simulink model "rocket_sim"  (R2023a)
settings: Solver=VariableStepAuto  StartTime=0.0  StopTime=480  RelTol=1e-3
undefined symbols (not defined in the file or in its folder): Earth, WGS84
libraries: simulink x55, slpidlib x10, aerolibconvert2 x7, matrix_library x4, aerolibasang x3, aerolibtransform2 x2, aerolibatmos2 x2, shared6dof x1, sharedtransform x1
(part 1 of 3)
settings Model: Creator=Administrator  LastModifiedBy=ROG

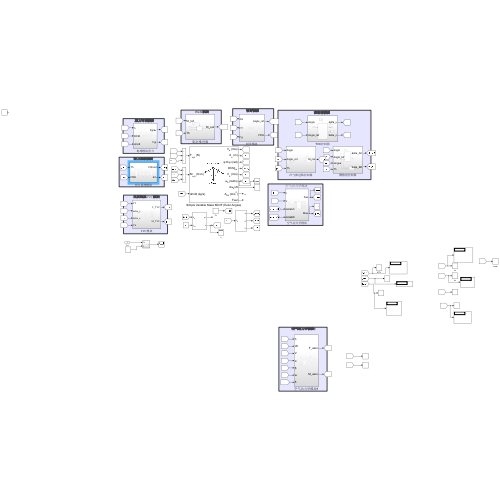
[thumbnail: Simulink's stored preview of the top-level diagram]
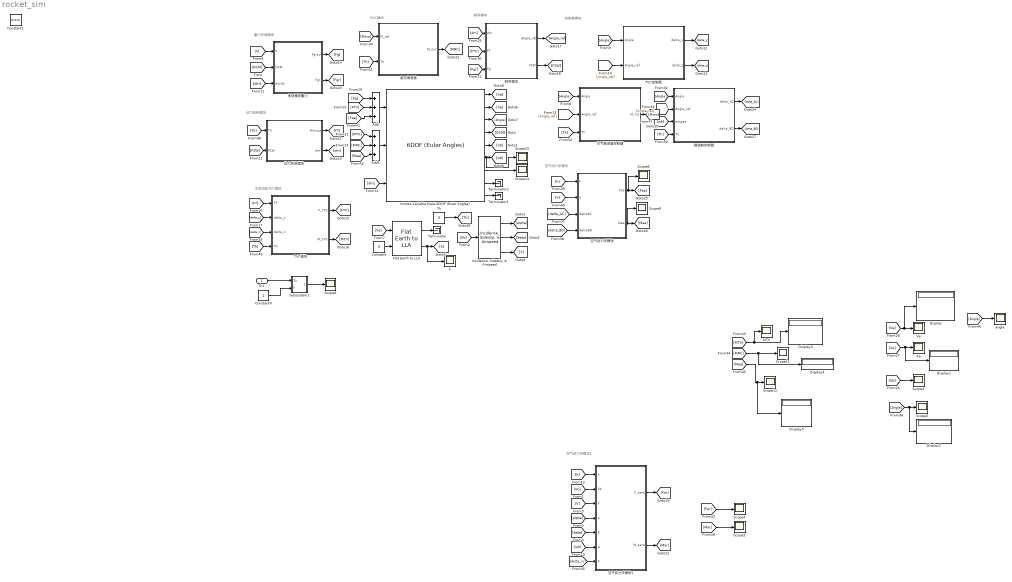
== system rocket_sim ==
  note: 空气动力学模块
  note: 控制器模块
  note: 空气动力学模块1
  note: 制导模块
  note: RCS模块
  note: 动力系统模块
  note: 重力环境模块
  note: 主发动机TVC模块
  Th1 : Inport
  Add : Sum  Inputs=+++
  Add1 : Sum  Inputs=+++
  Constant : Constant  Value=0
  Constant1 : Constant  Value=[0;0;0]
  Constant4 : Constant
  Display{,1..5} (6 alike) : Display
  Flat Earth to LLA : aerolibtransform2/Flat Earth to LLA  units=Metric (MKS)  ptype=Earth (WGS84)  F=1/298.257223563  R=6378137  refPosPort=off  LL0=[0 10]  psi=0
  "Incidence, Sideslip, & Airspeed" : aerolibasang/Incidence, Sideslip, & Airspeed
  MTV : Scope
  Scope{2..6,8..9,11..12,14..15} (11 alike) : Scope
  Simple Variable Mass 6DOF (Euler Angles) : shared6dof/6DOF (Euler Angles)  units=Metric (MKS)  mtype=Simple Variable  rep=Euler Angles  xme_0=[0 0 0]  Vm_0=[0 0 0]  eul_0=[0 pi/2 0]  pm_0=[0 0 0]  mass_0=549e3  mass_e=22.2e3  mass_f=549e3  inertia=eye(3)  inertia_e=6.06e4*eye(3)  inertia_f=149.9e4*eye(3)  k_quat=1.0  vre_flag=off  abi_flag=off  aMode=0  xme_statename=''  Vm_statename=''  eul_statename=''  quat_statename=''  pm_statename=''  mass_statename=''
      settings: LibrarySourceBlock=aerolib6dof2/Simple Variable Mass 6DOF (Euler Angles)
  Subsystem1 : Subsystem
  TVC控制器 : Subsystem
  TVC模块 : Subsystem
  Terminator : Terminator
  Terminator1 : Terminator
  Terminator2 : Terminator
  Th : Constant  Value=0
  Ve : Scope
  Xe : Scope
  angle : Scope
  h : Scope
  冷气推进器控制器 : Subsystem
  制导模块 : Subsystem
  动力系统模块 : Subsystem
  地球模块重力 : Subsystem
  姿态推进器 : Subsystem
  栅格舵控制器 : Subsystem
  空气动力学模块 : Subsystem
  空气动力学模块1 : Subsystem
  wires:
  [h] -> 地球模块重力/1(h)
  Simple Variable Mass 6DOF (Euler Angles)/4 -> [DCM]
  [DCM] -> 地球模块重力/2(DCM)
  Simple Variable Mass 6DOF (Euler Angles)/5 -> [Vb]
  [Vb] -> 空气动力学模块1/2(Vb)
  [Vb] -> "Incidence, Sideslip, & Airspeed"/1
  "Incidence, Sideslip, & Airspeed"/1 -> [alpha]
  "Incidence, Sideslip, & Airspeed"/2 -> [beta]
  "Incidence, Sideslip, & Airspeed"/3 -> [V]
  [alpha] -> 空气动力学模块1/4(α)
  [beta] -> 空气动力学模块1/5(β)
  [V] -> 空气动力学模块1/3(V)
  Flat Earth to LLA/1 -> Terminator/1
  Flat Earth to LLA/2 -> h/1, [h]
  Constant/1 -> Flat Earth to LLA/2
  Simple Variable Mass 6DOF (Euler Angles)/2 -> [Xe]
  [Xe] -> Flat Earth to LLA/1
  Simple Variable Mass 6DOF (Euler Angles)/3 -> [Angle]
  Simple Variable Mass 6DOF (Euler Angles)/1 -> [Ve]
  Simple Variable Mass 6DOF (Euler Angles)/6 -> Scope15/1, [wb]
  动力系统模块/2(dm) -> [dm]
  [dm] -> 地球模块重力/3(dm/dt)
  [dm] -> Simple Variable Mass 6DOF (Euler Angles)/3
  [h] -> 空气动力学模块1/1(h)
  [FT] -> TVC模块/1(FT)
  [delta_y] -> TVC模块/2(delta_y)
  [delta_z] -> TVC模块/3(delta_z)
  Add/1 -> Simple Variable Mass 6DOF (Euler Angles)/1
  Add1/1 -> Simple Variable Mass 6DOF (Euler Angles)/2
  地球模块重力/1(Fgrav) -> [Fg]
  [Fg] -> Add/1
  TVC模块/1(F_TVC) -> [FTV]
  TVC模块/2(M_TVC) -> [MTV]
  [FTV] -> Add/2
  [MTV] -> Add1/1
  动力系统模块/1(Fthrust) -> [FT]
  [wb] -> 空气动力学模块1/6(w)
  制导模块/1(Angle_ref) -> [Angle_ref]
  Simple Variable Mass 6DOF (Euler Angles)/9 -> Terminator1/1
  Simple Variable Mass 6DOF (Euler Angles)/8 -> Terminator2/1
  [Angle] -> TVC控制器/1(Angle)
  [Angle_ref] -> TVC控制器/2(Angle_ref)
  TVC控制器/2(delta_z) -> [delta_z]
  TVC控制器/1(delta_y) -> [delta_y]
  制导模块/2(FSW) -> [FSW]
  [FSW] -> 动力系统模块/2(FSW)
  空气动力学模块1/1(F_aero) -> [Far]
  空气动力学模块1/2(M_aero) -> [Mar]
  姿态推进器/1(M_out) -> [MRC]
  [Ve] -> Display/1, Ve/1
  [Xe] -> Display1/1, Xe/1
  [Vb] -> Scope2/1
  [MRC] -> Add1/2
  [dm] -> 制导模块/1(dm)
  [FTV] -> 制导模块/2(FT)
  [Fgr] -> 制导模块/3(Fg)
  地球模块重力/2(Fgr) -> [Fgr]
  [delta_ru] -> 空气动力学模块1/7(δ)
  [Angle] -> Display2/1, Scope3/1
  [Far] -> Scope4/1
  [Mar] -> Scope5/1
  冷气推进器控制器/1(M_rcs) -> [Mrcs]
  栅格舵控制器/1(delta_AC) -> [delta_AC]
  [Mrcs] -> 姿态推进器/1(M_ref)
  [Angle_ref] -> 冷气推进器控制器/2(Angle_ref)
  [Angle] -> 冷气推进器控制器/1(Angle)
  [Angle_ref] -> 栅格舵控制器/2(Angle_ref)
  [Angle] -> 栅格舵控制器/1(Angle)
  Constant4/1 -> Subsystem1/2(F)
  Th1/1 -> Subsystem1/1(Th)
  Subsystem1/1(Out1) -> Scope6/1
  [Faa] -> Add/3
  [Maa] -> Add1/3
  空气动力学模块/1(Faa) -> Scope8/1, [Faa]
  空气动力学模块/2(Maa) -> Scope9/1, [Maa]
  [h] -> 空气动力学模块/1(h)
  [V] -> 空气动力学模块/2(V)
  栅格舵控制器/2(delta_BD) -> [delta_BD]
  [MTV] -> MTV/1, Display3/1
  [MRC] -> Display4/1, Scope11/1
  [Maa] -> Display5/1, Scope12/1
  [delta_AC] -> 空气动力学模块/3(deltaAC)
  [delta_BD] -> 空气动力学模块/4(deltaBD)
  [Angle] -> angle/1
  Simple Variable Mass 6DOF (Euler Angles)/7 -> Scope14/1
  [wb] -> 栅格舵控制器/3(omgea)
  Th/1 -> [Th]
  [Th] -> 动力系统模块/1(Th)
  [Th] -> TVC模块/4(Th)
  [Th] -> 栅格舵控制器/4(Th)
  [Th] -> 姿态推进器/2(Th)
  [Th] -> 冷气推进器控制器/3(Th)

== system rocket_sim/Subsystem1 ==
  Th : Inport
  F : Inport  Port=2
  Constant4 : Constant  Value=0
  Step1 : Step  Time=200  SampleTime=0
  Step2 : Step  Time=480  SampleTime=0
  Switch : Switch  Criteria=u2 > Threshold  SaturateOnIntegerOverflow=off  InputSameDT=off
  Switch1 : Switch  Criteria=u2 > Threshold  SaturateOnIntegerOverflow=off  InputSameDT=off
  Switch2 : Switch  Criteria=u2 > Threshold  SaturateOnIntegerOverflow=off  InputSameDT=off
  故障 : Subsystem
  退化 : Subsystem
  Out1 : Outport
  wires:
  F/1 -> Switch2/2
  退化/1(Out1) -> Switch1/3, Switch/1
  Switch1/1 -> Switch/3
  Constant4/1 -> Switch2/1
  Switch2/1 -> Switch1/2
  Th/1 -> 故障/1(Th1), 退化/1(Th)
  Step2/1 -> Switch/2
  Switch/1 -> Out1/1
  Step1/1 -> Switch2/3
  故障/1(Out1) -> Switch1/1

== system rocket_sim/TVC控制器 ==
  Angle : Inport
  Angle_ref : Inport  Port=2
  Constant : Constant
  Scope : Scope
  Scope1 : Scope
  Subsystem : Subsystem
  delta_y : Outport
  delta_z : Outport  Port=2
  wires:
  Angle/1 -> Subsystem/1(Angle)
  Angle_ref/1 -> Subsystem/2(Angle_ref)
  Subsystem/1(delta_z) -> Scope/1, delta_z/1
  Subsystem/2(delta_y) -> Scope1/1, delta_y/1
  Constant/1 -> Subsystem/Enable

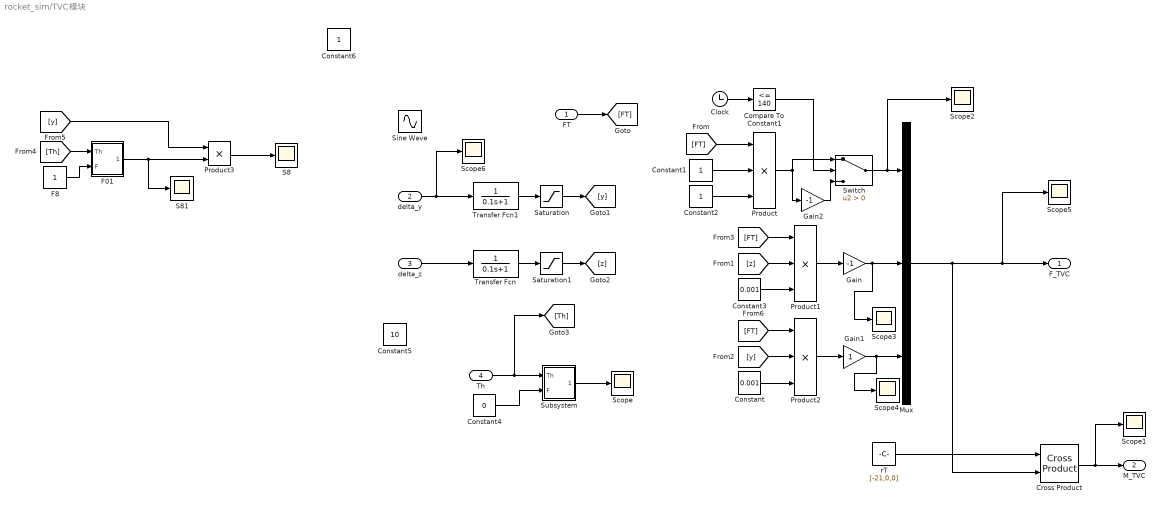
== system rocket_sim/TVC模块 ==
  FT : Inport
  delta_y : Inport  Port=2
  delta_z : Inport  Port=3
  Th : Inport  Port=4
  Clock : Clock
  Compare To Constant1 : simulink/Logic and Bit Operations/Compare To Constant  relop=<=  const=140  OutDataTypeStr=boolean
  Constant : Constant  Value=0.001
  Constant1 : Constant
  Constant2 : Constant
  Constant3 : Constant  Value=0.001
  Constant4 : Constant  Value=0
  Constant5 : Constant  Value=10
  Constant6 : Constant
  Cross Product : matrix_library/Cross Product
  F01 : Subsystem
  F8 : Constant
  Gain : Gain  Gain=-1
  Gain1 : Gain
  Gain2 : Gain  Gain=-1
  Mux : Mux  Inputs=3
  Product : Product  Inputs=3
  Product1 : Product  Inputs=3
  Product2 : Product  Inputs=3
  Product3 : Product
  S8 : Scope
  S81 : Scope
  Saturation : Saturate  UpperLimit=3  LowerLimit=-3
  Saturation1 : Saturate  UpperLimit=3  LowerLimit=-3
  Scope{,1..6} (7 alike) : Scope
  Sine Wave : Sin  SampleTime=0
  Subsystem : Subsystem
  Switch : Switch  Criteria=u2 > Threshold  SaturateOnIntegerOverflow=off  InputSameDT=off
  Transfer Fcn : TransferFcn  Denominator=[0.1 1]
  Transfer Fcn1 : TransferFcn  Denominator=[0.1 1]
  rT : Constant  Value=[-21,0,0]
  F_TVC : Outport
  M_TVC : Outport  Port=2
  wires:
  FT/1 -> [FT]
  [FT] -> Product/1
  Constant2/1 -> Product/3
  [FT] -> Product1/1
  [FT] -> Product2/1
  Constant/1 -> Product2/3
  Product1/1 -> Gain/1
  Product2/1 -> Gain1/1
  Gain/1 -> Scope3/1, Mux/2
  Gain1/1 -> Scope4/1, Mux/3
  Mux/1 -> Cross Product/2, Scope5/1, F_TVC/1
  rT/1 -> Cross Product/1
  Cross Product/1 -> Scope1/1, M_TVC/1
  delta_z/1 -> Transfer Fcn/1
  Transfer Fcn/1 -> Saturation1/1
  delta_y/1 -> Scope6/1, Transfer Fcn1/1
  Transfer Fcn1/1 -> Saturation/1
  Constant1/1 -> Product/2
  Saturation/1 -> [y]
  Saturation1/1 -> [z]
  [z] -> Product1/2
  [y] -> Product2/2
  Constant3/1 -> Product1/3
  Th/1 -> [Th], Subsystem/1(Th)
  Subsystem/1(Out1) -> Scope/1
  Constant4/1 -> Subsystem/2(F)
  Switch/1 -> Scope2/1, Mux/1
  Product/1 -> Gain2/1, Switch/1
  Gain2/1 -> Switch/3
  Clock/1 -> Compare To Constant1/1
  Compare To Constant1/1 -> Switch/2
  [Th] -> F01/1(Th)
  F01/1(Out1) -> S81/1, Product3/2
  F8/1 -> F01/2(F)
  [y] -> Product3/1
  Product3/1 -> S8/1

== system rocket_sim/冷气推进器控制器 ==
  Angle : Inport
  Angle_ref : Inport  Port=2
  Th : Inport  Port=3
  Constant : Constant
  Constant4 : Constant  Value=0
  Scope : Scope
  Subsystem : Subsystem
  Subsystem1 : Subsystem
  M_rcs : Outport
  wires:
  Angle/1 -> Subsystem/1(Angle)
  Angle_ref/1 -> Subsystem/2(Angle_ref)
  Subsystem/1(M_rcs) -> M_rcs/1
  Th/1 -> Subsystem1/1(Th)
  Subsystem1/1(Out1) -> Scope/1
  Constant4/1 -> Subsystem1/2(F)
  Constant/1 -> Subsystem/Enable

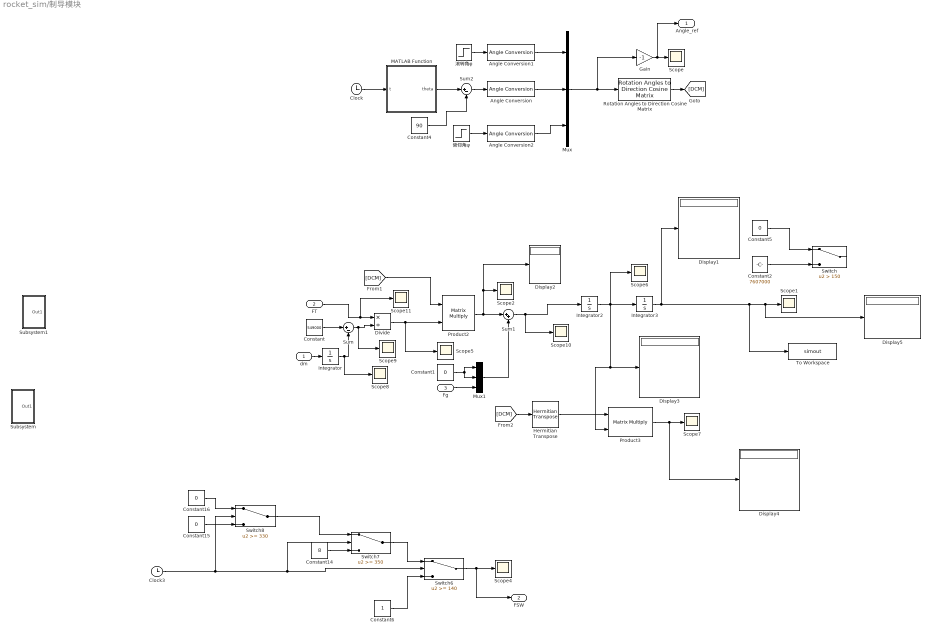
== system rocket_sim/制导模块 ==
  dm : Inport
  FT : Inport  Port=2
  Fg : Inport  Port=3
  Angle Conversion : aerolibconvert2/Angle Conversion  IU=deg  OU=rad
  Angle Conversion1 : aerolibconvert2/Angle Conversion  IU=deg  OU=rad
  Angle Conversion2 : aerolibconvert2/Angle Conversion  IU=deg  OU=rad
  Clock : Clock
  Clock3 : Clock
  Constant : Constant  Value=549000
  Constant{1,5,15..16} (4 alike) : Constant  Value=0
  Constant14 : Constant  Value=8
  Constant2 : Constant  Value=7607000
  Constant4 : Constant  Value=90
  Constant6 : Constant
  Display{1..5} (5 alike) : Display
  Divide : Product  Inputs=*/
  Gain : Gain  Gain=-1
  Hermitian Transpose : matrix_library/Hermitian Transpose
      settings: LibrarySourceBlock=|
      | simulink/Matrix
      | Operations/Hermitian Transpose
  Integrator : Integrator
  Integrator2 : Integrator
  Integrator3 : Integrator
  MATLAB Function : MATLAB Function  TreatAsAtomicUnit=on
  Mux : Mux  Inputs=3
  Mux1 : Mux  Inputs=3
  Product2 : Product  Multiplication=Matrix(*)
  Product3 : Product  Multiplication=Matrix(*)
  Rotation Angles to Direction Cosine Matrix : sharedtransform/Rotation Angles to Direction Cosine Matrix  rotationOrder=XYZ  aMode=aMode
  Scope{,1..2,4..11} (11 alike) : Scope
  Subsystem : Subsystem
  Subsystem1 : Subsystem
  Sum : Sum  Inputs=|+-
  Sum1 : Sum  Inputs=|++
  Sum2 : Sum  Inputs=|+-
  Switch : Switch  Criteria=u2 > Threshold  Threshold=150  SaturateOnIntegerOverflow=off  InputSameDT=off
  Switch6 : Switch  Threshold=140  SaturateOnIntegerOverflow=off  InputSameDT=off
  Switch7 : Switch  Threshold=350  SaturateOnIntegerOverflow=off  InputSameDT=off
  Switch8 : Switch  Threshold=330  SaturateOnIntegerOverflow=off  InputSameDT=off
  To Workspace : ToWorkspace  VariableName=simout  SaveFormat=Timeseries  SampleTime=-1
  俯仰角ψ : Step  Time=0  After=0  SampleTime=0
  滚转角φ : Step  Time=0  After=0  SampleTime=0
  Angle_ref : Outport
  FSW : Outport  Port=2
  wires:
  Constant5/1 -> Switch/1
  Constant2/1 -> Switch/3
  Clock/1 -> MATLAB Function/1(t)
  滚转角φ/1 -> Angle Conversion1/1
  俯仰角ψ/1 -> Angle Conversion2/1
  Angle Conversion1/1 -> Mux/1
  Angle Conversion/1 -> Mux/2
  Angle Conversion2/1 -> Mux/3
  Mux/1 -> Gain/1, Rotation Angles to Direction Cosine Matrix/1
  Rotation Angles to Direction Cosine Matrix/1 -> [DCM]
  Integrator2/1 -> Scope6/1, Display3/1, Product3/2, Integrator3/1
  Integrator3/1 -> Display1/1, To Workspace/1, Display5/1, Scope1/1
  MATLAB Function/1(theta) -> Sum2/1
  Sum2/1 -> Angle Conversion/1
  Product2/1 -> Display2/1, Scope2/1, Sum1/1
  Divide/1 -> Scope5/1, Product2/2
  Constant4/1 -> Sum2/2
  Product3/1 -> Display4/1, Scope7/1
  [DCM] -> Product2/1
  [DCM] -> Hermitian Transpose/1
  Hermitian Transpose/1 -> Product3/1
  Clock3/1 -> Switch8/2, Switch7/2, Switch6/2
  Constant6/1 -> Switch6/3
  Switch7/1 -> Switch6/1
  Switch8/1 -> Switch7/1
  Constant14/1 -> Switch7/3
  Constant15/1 -> Switch8/3
  Constant16/1 -> Switch8/1
  Switch6/1 -> FSW/1, Scope4/1
  Sum/1 -> Scope9/1, Divide/2
  Constant/1 -> Sum/1
  dm/1 -> Integrator/1
  Integrator/1 -> Scope8/1, Sum/2
  FT/1 -> Scope11/1, Divide/1
  Sum1/1 -> Scope10/1, Integrator2/1
  Fg/1 -> Mux1/3
  Constant1/1 -> Mux1/1, Mux1/2
  Mux1/1 -> Sum1/2
  Gain/1 -> Angle_ref/1, Scope/1

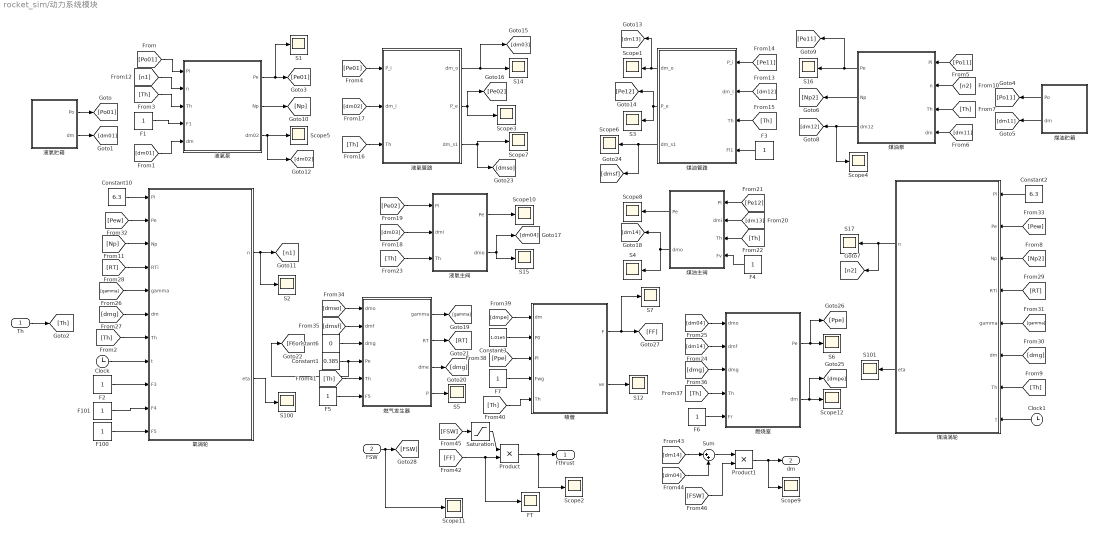
== system rocket_sim/动力系统模块 ==
  Th : Inport
  FSW : Inport  Port=2
  Clock : Clock
  Clock1 : Clock
  Constant1 : Constant  Value=0.385
  Constant10 : Constant  Value=6.3
  Constant2 : Constant  Value=6.3
  Constant3 : Constant  Value=1.01e5
  Constant6 : Constant  Value=0
  F{1..7,100..101} (9 alike) : Constant
  FT : Scope
  Product : Product
  Product1 : Product
  S{1..7,12,14..17,100..101} (14 alike) : Scope
  Saturation : Saturate  UpperLimit=9  LowerLimit=0
  Scope{1..12} (12 alike) : Scope
  Sum : Sum  Inputs=|++
  喷管 : Subsystem
  氧涡轮 : Subsystem
  液氧主阀 : Subsystem
  液氧泵 : Subsystem
  液氧管路 : Subsystem
  液氧贮箱 : Subsystem
  煤油主阀 : Subsystem
  煤油泵 : Subsystem
  煤油涡轮 : Subsystem
  煤油管路 : Subsystem
  煤油贮箱 : Subsystem
  燃气发生器 : Subsystem
  燃烧室 : Subsystem
  Fthrust : Outport
  dm : Outport  Port=2
  wires:
  [dmg] -> 氧涡轮/6(dm)
  液氧泵/1(Pe) -> [Pe01], S1/1
  Clock/1 -> 氧涡轮/8(t)
  F1/1 -> 液氧泵/4(F1)
  [n1] -> 液氧泵/2(n)
  F101/1 -> 氧涡轮/10(F4)
  Constant10/1 -> 氧涡轮/1(Pi)
  液氧泵/2(Np) -> [Np]
  F100/1 -> 氧涡轮/11(F5)
  氧涡轮/2(eta) -> S100/1
  F2/1 -> 氧涡轮/9(F3)
  [RT] -> 氧涡轮/4(RTi)
  [Np] -> 氧涡轮/3(Np)
  氧涡轮/1(n) -> [n1], S2/1
  液氧贮箱/1(Po) -> [Po01]
  液氧贮箱/2(dm) -> [dm01]
  [Po01] -> 液氧泵/1(Pi)
  [dm01] -> 液氧泵/5(dm)
  Th/1 -> [Th]
  [Th] -> 氧涡轮/7(Th)
  [Th] -> 液氧泵/3(Th)
  煤油贮箱/2(dm) -> [dm11]
  煤油贮箱/1(Po) -> [Po11]
  [Po11] -> 煤油泵/1(Pi)
  [dm11] -> 煤油泵/4(dm)
  [Th] -> 煤油泵/3(Th)
  煤油泵/1(Pe) -> [Pe11], S16/1
  煤油泵/2(Np) -> [Np2]
  Clock1/1 -> 煤油涡轮/8(t)
  [gamma] -> 煤油涡轮/5(gamma)
  Constant2/1 -> 煤油涡轮/1(Pi)
  [Np2] -> 煤油涡轮/3(Np)
  [RT] -> 煤油涡轮/4(RTi)
  [dmg] -> 煤油涡轮/6(dm)
  [Th] -> 煤油涡轮/7(Th)
  煤油涡轮/1(n) -> [n2], S17/1
  煤油涡轮/2(eta) -> S101/1
  [n2] -> 煤油泵/2(n)
  煤油泵/3(dm12) -> Scope4/1, [dm12]
  液氧泵/3(dm02) -> [dm02], Scope5/1
  [Th] -> 煤油管路/3(Th)
  [dm12] -> 煤油管路/2(dm_i)
  [Pe11] -> 煤油管路/1(P_i)
  F3/1 -> 煤油管路/4(Fl1)
  煤油管路/1(dm_o) -> [dm13], Scope1/1
  煤油管路/2(P_e) -> [Pe12], S3/1
  [Pe01] -> 液氧管路/1(P_i)
  [Th] -> 液氧管路/3(Th)
  [dm02] -> 液氧管路/2(dm_i)
  液氧管路/1(dm_o) -> [dm03], S14/1
  液氧管路/2(P_e) -> [Pe02], Scope3/1
  煤油管路/3(dm_s1) -> [dmsf], Scope6/1
  液氧管路/3(dm_s1) -> [dmso], Scope7/1
  [Th] -> 煤油主阀/3(Th)
  [Pe12] -> 煤油主阀/1(Pi)
  [dm13] -> 煤油主阀/2(dmi)
  煤油主阀/1(Pe) -> Scope8/1
  煤油主阀/2(dmo) -> [dm14], S4/1
  F4/1 -> 煤油主阀/4(Fv)
  [dm03] -> 液氧主阀/2(dmi)
  [Pe02] -> 液氧主阀/1(Pi)
  [Th] -> 液氧主阀/3(Th)
  液氧主阀/1(Pe) -> Scope10/1
  液氧主阀/2(dmo) -> [dm04], S15/1
  Constant6/1 -> 燃气发生器/3(dmg)
  燃气发生器/1(gamma) -> [gamma]
  [gamma] -> 氧涡轮/5(gamma)
  燃气发生器/3(dme) -> [dmg]
  燃气发生器/2(RT) -> [RT]
  Constant1/1 -> [Pew], 燃气发生器/4(Pe)
  [Pew] -> 氧涡轮/2(Pe)
  [Pew] -> 煤油涡轮/2(Pe)
  燃气发生器/4(P) -> S5/1
  [dmso] -> 燃气发生器/1(dmo)
  [dmsf] -> 燃气发生器/2(dmf)
  [dm04] -> 燃烧室/1(dmo)
  [dm14] -> 燃烧室/2(dmf)
  [dmg] -> 燃烧室/3(dmg)
  [Th] -> 燃烧室/4(Th)
  F6/1 -> 燃烧室/5(Fr)
  燃烧室/1(Pe) -> [Ppe], S6/1
  燃烧室/2(dm) -> [dmpe], Scope12/1
  [dmpe] -> 喷管/1(dm)
  Constant3/1 -> 喷管/2(P0)
  [Ppe] -> 喷管/3(Pi)
  喷管/1(F) -> [FF], S7/1
  喷管/2(ve) -> S12/1
  F7/1 -> 喷管/4(Fwg)
  [Th] -> 喷管/5(Th)
  [Th] -> 燃气发生器/5(Th)
  F5/1 -> 燃气发生器/6(F5)
  [dm14] -> Sum/1
  [dm04] -> Sum/2
  FSW/1 -> Scope11/1, [FSW]
  [FF] -> FT/1, Product/2
  Product/1 -> Scope2/1, Fthrust/1
  Sum/1 -> Product1/1
  Product1/1 -> Scope9/1, dm/1
  [FSW] -> Product1/2
  [FSW] -> Saturation/1
  Saturation/1 -> Product/1

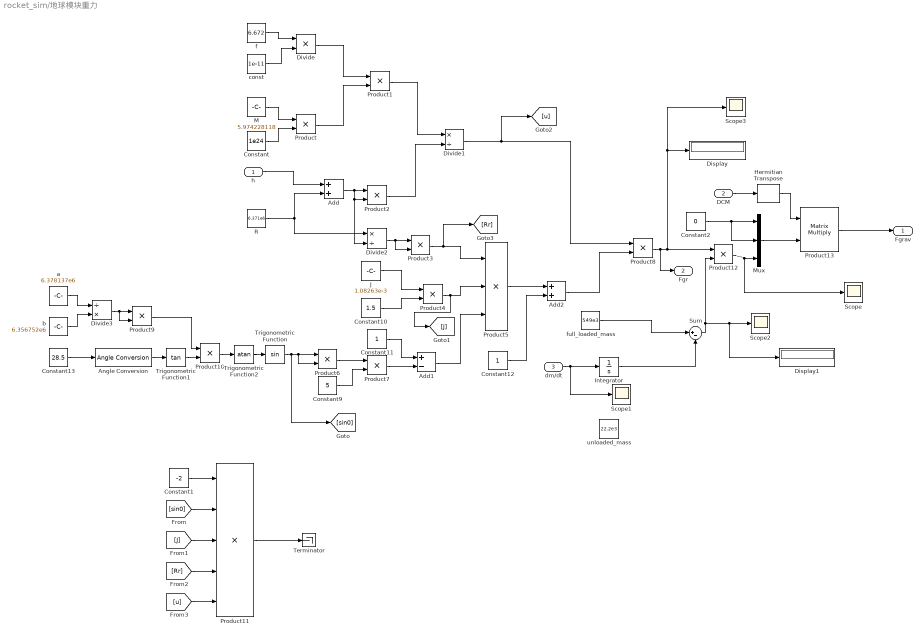
== system rocket_sim/地球模块重力 ==
  h : Inport
  DCM : Inport  Port=2
  dm/dt : Inport  Port=3
  Add : Sum
  Add1 : Sum  Inputs=+-
  Add2 : Sum
  Angle Conversion : aerolibconvert2/Angle Conversion  IU=deg  OU=rad
  Constant : Constant  Value=1e24
  Constant1 : Constant  Value=-2
  Constant10 : Constant  Value=1.5
  Constant11 : Constant
  Constant12 : Constant
  Constant13 : Constant  Value=28.5
  Constant2 : Constant  Value=0
  Constant9 : Constant  Value=5
  Display : Display
  Display1 : Display
  Divide : Product  Inputs=**
  Divide1 : Product  Inputs=*/
  Divide2 : Product  Inputs=*/
  Divide3 : Product  Inputs=/*
  Hermitian Transpose : matrix_library/Hermitian Transpose
      settings: LibrarySourceBlock=|
      | simulink/Matrix
      | Operations/Hermitian Transpose
  Integrator : Integrator
  J : Constant  Value=1.08263e-3
  M : Constant  Value=5.974228118
  Mux : Mux  Inputs=3
  Product{,1..4,6..10,12} (11 alike) : Product
  Product11 : Product  Inputs=5
  Product13 : Product  Multiplication=Matrix(*)
  Product5 : Product  Inputs=3
  R : Constant  Value=6.371e6
  Scope{,1..3} (4 alike) : Scope
  Sum : Sum  Inputs=|+-
  Terminator : Terminator
  Trigonometric Function : Trigonometry
  Trigonometric Function1 : Trigonometry  Operator=tan
  Trigonometric Function2 : Trigonometry  Operator=atan
  a : Constant  Value=6.378137e6
  b : Constant  Value=6.356752e6
  const : Constant  Value=1e-11
  f : Constant  Value=6.672
  full_loaded_mass : Constant  Value=549e3
  unloaded_mass : Constant  Value=22.2e3
  Fgrav : Outport
  Fgr : Outport  Port=2
  wires:
  R/1 -> Divide2/1, Add/2
  Constant13/1 -> Angle Conversion/1
  Trigonometric Function2/1 -> Trigonometric Function/1
  Divide3/1 -> Product9/2, Product9/1
  Angle Conversion/1 -> Trigonometric Function1/1
  Constant12/1 -> Add2/2
  Constant10/1 -> Product4/2
  Product9/1 -> Product10/1
  Divide1/1 -> [u], Product8/1
  Constant/1 -> Product/2
  b/1 -> Divide3/2
  Product/1 -> Product1/2
  Trigonometric Function/1 -> [sin0], Product6/2, Product6/1
  Constant9/1 -> Product7/2
  h/1 -> Add/1
  Product4/1 -> [J], Product5/2
  Add/1 -> Divide2/2, Product2/2, Product2/1
  Divide/1 -> Product1/1
  Constant11/1 -> Add1/1
  const/1 -> Divide/2
  f/1 -> Divide/1
  Product7/1 -> Add1/2
  Product2/1 -> Divide1/2
  Product1/1 -> Divide1/1
  a/1 -> Divide3/1
  Product5/1 -> Add2/1
  Product10/1 -> Trigonometric Function2/1
  Divide2/1 -> Product3/2, Product3/1
  Product6/1 -> Product7/1
  Trigonometric Function1/1 -> Product10/2
  Add2/1 -> Product8/2
  M/1 -> Product/1
  Add1/1 -> Product5/3
  J/1 -> Product4/1
  Product3/1 -> [Rr], Product5/1
  Constant1/1 -> Product11/1
  [sin0] -> Product11/2
  [J] -> Product11/3
  [Rr] -> Product11/4
  [u] -> Product11/5
  Product11/1 -> Terminator/1
  dm/dt/1 -> Scope1/1, Integrator/1
  full_loaded_mass/1 -> Sum/1
  Integrator/1 -> Sum/2
  Sum/1 -> Product12/2, Display1/1, Scope2/1
  Product8/1 -> Fgr/1, Scope3/1, Display/1, Product12/1
  Product12/1 -> Mux/3, Scope/1
  Mux/1 -> Product13/2
  Constant2/1 -> Mux/2, Mux/1
  DCM/1 -> Hermitian Transpose/1
  Hermitian Transpose/1 -> Product13/1
  Product13/1 -> Fgrav/1

== system rocket_sim/姿态推进器 ==
  M_ref : Inport
  Th : Inport  Port=2
  Constant : Constant
  RCS : Subsystem
  M_out : Outport
  wires:
  M_ref/1 -> RCS/1(M_ref)
  RCS/1(M_out) -> M_out/1
  Constant/1 -> RCS/Enable
  Th/1 -> RCS/2(Th)

== system rocket_sim/栅格舵控制器 ==
  Angle : Inport
  Angle_ref : Inport  Port=2
  omgea : Inport  Port=3
  Th : Inport  Port=4
  Constant : Constant
  Constant1 : Constant  Value=0
  Subsystem1 : Subsystem
  Terminator : Terminator
  Terminator1 : Terminator
  栅格舵 : Subsystem
  delta_AC : Outport
  delta_BD : Outport  Port=2
  wires:
  Angle/1 -> Subsystem1/1(In1), 栅格舵/1(Angle)
  Angle_ref/1 -> Subsystem1/2(In2), 栅格舵/2(Angle_ref)
  栅格舵/1(delta_AC) -> delta_AC/1
  Constant/1 -> 栅格舵/Enable
  栅格舵/2(delta_BD) -> delta_BD/1
  omgea/1 -> Subsystem1/3(omgea)
  Constant1/1 -> Subsystem1/Enable
  Subsystem1/1(delta_AC1) -> Terminator/1
  Subsystem1/2(delta_BD1) -> Terminator1/1
  Th/1 -> 栅格舵/3(Th)

== system rocket_sim/空气动力学模块 ==
  h : Inport
  V : Inport  Port=2
  deltaAC : Inport  Port=3
  deltaBD : Inport  Port=4
  ISA Atmosphere Model : aerolibatmos2/ISA Atmosphere Model  custom=off  g=9.80665  gamma=1.4  R=287.0531  L=0.0065  h_trop=11000  h_strat=20000  rho0=1.225  P0=101325  T0=288.15  h0=0
  MATLAB Function : MATLAB Function  TreatAsAtomicUnit=on
  Scope1 : Scope
  Scope8 : Scope
  Scope9 : Scope
  Terminator : Terminator
  Terminator1 : Terminator
  Terminator2 : Terminator
  Faa : Outport
  Maa : Outport  Port=2
  wires:
  MATLAB Function/1(F_a) -> Scope8/1, Faa/1
  ISA Atmosphere Model/4 -> MATLAB Function/1(rho)
  V/1 -> MATLAB Function/2(V)
  h/1 -> ISA Atmosphere Model/1
  MATLAB Function/2(M_a) -> Scope9/1, Maa/1
  ISA Atmosphere Model/1 -> Terminator/1
  ISA Atmosphere Model/2 -> Terminator1/1
  ISA Atmosphere Model/3 -> Terminator2/1
  deltaAC/1 -> MATLAB Function/3(deltaAC)
  deltaBD/1 -> MATLAB Function/4(deltaBD)
  MATLAB Function/3(q) -> Scope1/1

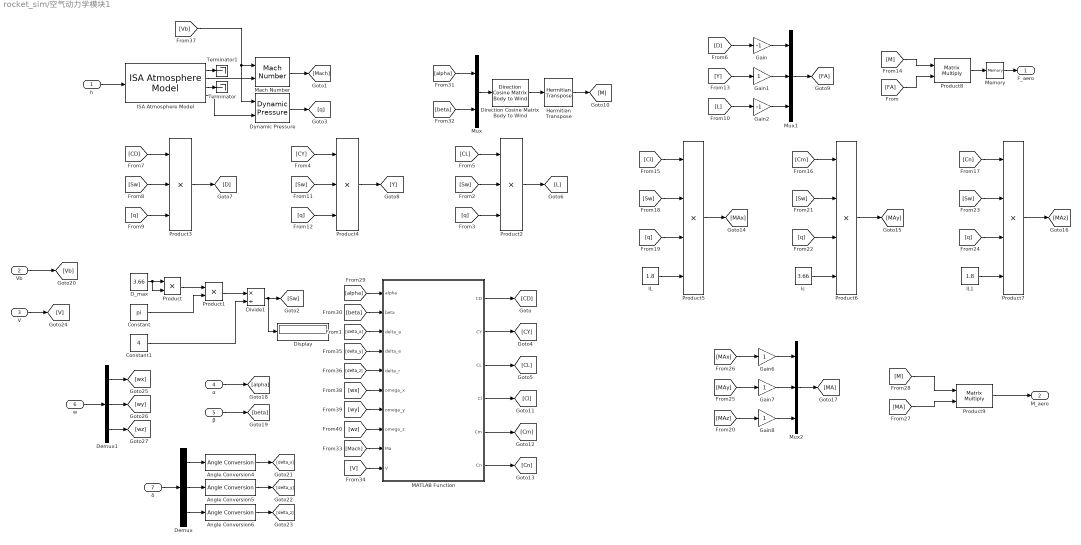
== system rocket_sim/空气动力学模块1 ==
  h : Inport
  Vb : Inport  Port=2
  V : Inport  Port=3
  α : Inport  Port=4
  β : Inport  Port=5
  w : Inport  Port=6
  δ : Inport  Port=7
  Angle Conversion4 : aerolibconvert2/Angle Conversion  IU=deg  OU=rad
  Angle Conversion5 : aerolibconvert2/Angle Conversion  IU=deg  OU=rad
  Angle Conversion6 : aerolibconvert2/Angle Conversion  IU=deg  OU=rad
  Constant : Constant  Value=pi
  Constant1 : Constant  Value=4
  D_max : Constant  Value=3.66
  Demux : Demux  Outputs=3
  Demux1 : Demux  Outputs=3
  Direction Cosine Matrix Body to Wind : aerolibtransform2/Direction Cosine Matrix Body to Wind
  Display : Display
  Divide1 : Product  Inputs=*/
  Dynamic Pressure : aerolibasang/Dynamic Pressure
  Gain : Gain  Gain=-1
  Gain{1,6..8} (4 alike) : Gain
  Gain2 : Gain  Gain=-1
  Hermitian Transpose : matrix_library/Hermitian Transpose
      settings: LibrarySourceBlock=|
      | simulink/Matrix
      | Operations/Hermitian Transpose
  ISA Atmosphere Model : aerolibatmos2/ISA Atmosphere Model  custom=off  g=9.80665  gamma=1.4  R=287.0531  L=0.0065  h_trop=11000  h_strat=20000  rho0=1.225  P0=101325  T0=288.15  h0=0
  MATLAB Function : MATLAB Function  TreatAsAtomicUnit=on
  Mach Number : aerolibasang/Mach Number
  Memory : Memory
  Mux : Mux  Inputs=2
  Mux1 : Mux  Inputs=3
  Mux2 : Mux  Inputs=3
  Product : Product
  Product1 : Product
  Product2 : Product  Inputs=3
  Product3 : Product  Inputs=3
  Product4 : Product  Inputs=3
  Product5 : Product  Inputs=4
  Product6 : Product  Inputs=4
  Product7 : Product  Inputs=4
  Product8 : Product  Multiplication=Matrix(*)
  Product9 : Product  Multiplication=Matrix(*)
  Terminator : Terminator
  Terminator1 : Terminator
  lL : Constant  Value=1.8
  lL1 : Constant  Value=1.8
  lc : Constant  Value=3.66
  F_aero : Outport
  M_aero : Outport  Port=2
  wires:
  [Cn] -> Product7/1
  Product/1 -> Product1/1
  ISA Atmosphere Model/4 -> Dynamic Pressure/2
  Constant/1 -> Product1/2
  [q] -> Product7/3
  Mux/1 -> Direction Cosine Matrix Body to Wind/1
  MATLAB Function/4(Cl) -> [Cl]
  Product2/1 -> [L]
  [q] -> Product6/3
  lL/1 -> Product5/4
  Product5/1 -> [MAx]
  Gain1/1 -> Mux1/2
  [V] -> MATLAB Function/10(V)
  Angle Conversion4/1 -> [delta_x]
  lc/1 -> Product6/4
  lL1/1 -> Product7/4
  β/1 -> [beta]
  Gain8/1 -> Mux2/3
  MATLAB Function/6(Cn) -> [Cn]
  [Sw] -> Product2/2
  Divide1/1 -> Display/1, [Sw]
  [q] -> Product4/3
  [M] -> Product9/1
  Hermitian Transpose/1 -> [M]
  [MAz] -> Gain8/1
  Gain6/1 -> Mux2/1
  [Sw] -> Product5/2
  [q] -> Product2/3
  D_max/1 -> Product/2, Product/1
  [D] -> Gain/1
  [Cm] -> Product6/1
  [L] -> Gain2/1
  Product3/1 -> [D]
  [Sw] -> Product3/2
  ISA Atmosphere Model/3 -> Terminator/1
  Product7/1 -> [MAz]
  Gain/1 -> Mux1/1
  [Y] -> Gain1/1
  δ/1 -> Demux/1
  Mux2/1 -> [MA]
  Product1/1 -> Divide1/1
  Dynamic Pressure/1 -> [q]
  [q] -> Product3/3
  Gain7/1 -> Mux2/2
  [FA] -> Product8/2
  Angle Conversion6/1 -> [delta_z]
  [MAx] -> Gain6/1
  [Cl] -> Product5/1
  h/1 -> ISA Atmosphere Model/1
  ISA Atmosphere Model/1 -> Terminator1/1
  Direction Cosine Matrix Body to Wind/1 -> Hermitian Transpose/1
  [MAy] -> Gain7/1
  [Sw] -> Product7/2
  [CL] -> Product2/1
  [Sw] -> Product4/2
  Product4/1 -> [Y]
  MATLAB Function/1(CD) -> [CD]
  MATLAB Function/2(CY) -> [CY]
  MATLAB Function/5(Cm) -> [Cm]
  Product6/1 -> [MAy]
  [Mach] -> MATLAB Function/9(Ma)
  Mach Number/1 -> [Mach]
  Gain2/1 -> Mux1/3
  [q] -> Product5/3
  ISA Atmosphere Model/2 -> Mach Number/2
  [MA] -> Product9/2
  Mux1/1 -> [FA]
  [alpha] -> MATLAB Function/1(alpha)
  α/1 -> [alpha]
  [delta_z] -> MATLAB Function/5(delta_r)
  [Sw] -> Product6/2
  MATLAB Function/3(CL) -> [CL]
  Demux/2 -> Angle Conversion5/1
  Constant1/1 -> Divide1/2
  Angle Conversion5/1 -> [delta_y]
  [beta] -> MATLAB Function/2(beta)
  [M] -> Product8/1
  [CD] -> Product3/1
  [alpha] -> Mux/1
  [CY] -> Product4/1
  Demux/1 -> Angle Conversion4/1
  Demux/3 -> Angle Conversion6/1
  [beta] -> Mux/2
  Vb/1 -> [Vb]
  V/1 -> [V]
  [Vb] -> Dynamic Pressure/1, Mach Number/1
  w/1 -> Demux1/1
  Demux1/1 -> [wx]
  Demux1/2 -> [wy]
  Demux1/3 -> [wz]
  [wx] -> MATLAB Function/6(omega_x)
  [wy] -> MATLAB Function/7(omega_y)
  [wz] -> MATLAB Function/8(omega_z)
  [delta_y] -> MATLAB Function/4(delta_e)
  [delta_x] -> MATLAB Function/3(delta_a)
  Memory/1 -> F_aero/1
  Product8/1 -> Memory/1
  Product9/1 -> M_aero/1

== system rocket_sim/Subsystem1/故障 ==
  Th1 : Inport
  Band-Limited White Noise : simulink/Sources/Band-Limited White Noise  Cov=[0.1]  Ts=0.1  seed=[23341]
  Clock : Clock
  Constant : Constant
  Constant5 : Constant  Value=2
  Gain : Gain  Gain=-1.2153e-04
  Gain3 : Gain  Gain=0.0001
  Integrator : Integrator
  Product3 : Product
  Sum : Sum  Inputs=|+++
  Sum1 : Sum  Inputs=|++
  Out1 : Outport
  wires:
  Product3/1 -> Out1/1
  Sum1/1 -> Gain/1
  Gain3/1 -> Sum/2
  Constant5/1 -> Product3/1
  Integrator/1 -> Gain3/1
  Clock/1 -> Sum1/1
  Sum/1 -> Product3/2
  Band-Limited White Noise/1 -> Integrator/1
  Th1/1 -> Sum1/2
  Constant/1 -> Sum/3
  Gain/1 -> Sum/1

== system rocket_sim/Subsystem1/退化 ==
  Th : Inport
  Band-Limited White Noise : simulink/Sources/Band-Limited White Noise  Cov=[0.1]  Ts=0.1  seed=[23341]
  Clock : Clock
  Constant : Constant
  Constant4 : Constant  Value=16
  Gain : Gain  Gain=-1.2153e-04
  Gain3 : Gain  Gain=0.001
  Integrator : Integrator
  Product3 : Product
  Scope : Scope
  Sum : Sum  Inputs=|+++
  Sum1 : Sum  Inputs=|++
  Out1 : Outport
  wires:
  Clock/1 -> Sum1/1
  Band-Limited White Noise/1 -> Integrator/1
  Gain3/1 -> Sum/2
  Constant4/1 -> Product3/1
  Th/1 -> Sum1/2
  Integrator/1 -> Gain3/1
  Sum/1 -> Scope/1, Product3/2
  Product3/1 -> Out1/1
  Sum1/1 -> Gain/1
  Gain/1 -> Sum/1
  Constant/1 -> Sum/3

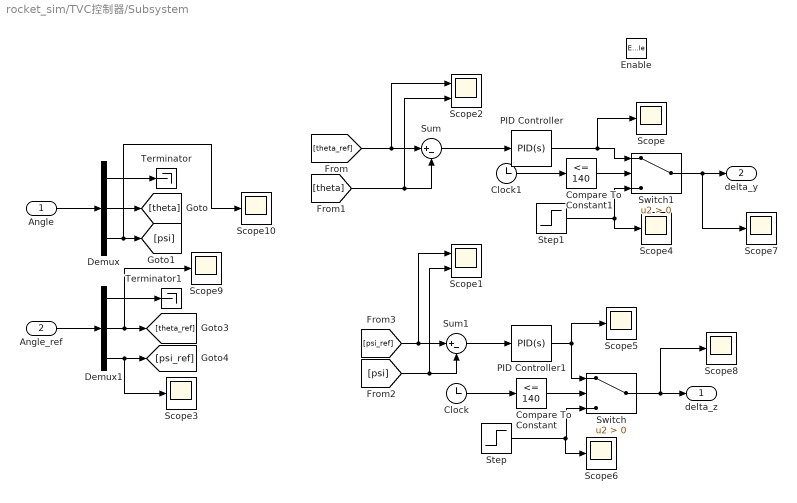
== system rocket_sim/TVC控制器/Subsystem ==
  Angle : Inport
  Angle_ref : Inport  Port=2
  Enable : EnablePort
  Clock : Clock
  Clock1 : Clock
  Compare To Constant : simulink/Logic and Bit Operations/Compare To Constant  relop=<=  const=140  OutDataTypeStr=boolean
  Compare To Constant1 : simulink/Logic and Bit Operations/Compare To Constant  relop=<=  const=140  OutDataTypeStr=boolean
  Demux : Demux  Outputs=3
  Demux1 : Demux  Outputs=3
  PID Controller : slpidlib/PID Controller  Controller=PID  Form=Parallel  TimeDomain=Continuous-time  UseExternalTs=off  SampleTime=-1  IntegratorMethod=Forward Euler  FilterMethod=Forward Euler  ControllerParametersSource=internal  P=10  I=0  UseKiTs=off  D=0  N=100  UseFilter=on  TunerSelectOption=Transfer Function Based (PID Tuner App)  InitialConditionSource=internal  InitialConditionForIntegrator=0  InitialConditionForFilter=0  DifferentiatorICPrevScaledInput=0  ExternalReset=none  TrackingMode=off  Kt=1  LimitOutput=off  SatLimitsSource=internal  UpperSaturationLimit=inf  LowerSaturationLimit=-inf  LinearizeAsGain=on  AntiWindupMode=none  Kb=1  LimitIntegrator=off  UpperIntegratorSaturationLimit=inf  LowerIntegratorSaturationLimit=-inf  POutMin=[]  POutMax=[]  IOutMin=[]  IOutMax=[]  DOutMin=[]  DOutMax=[]  NOutMin=[]  NOutMax=[]  SumOutMin=[]  SumOutMax=[]  SaturationOutMin=[]  SaturationOutMax=[]  PParamMin=[]  PParamMax=[]  IParamMin=[]  IParamMax=[]  DParamMin=[]  DParamMax=[]  NParamMin=[]  NParamMax=[]  KbParamMin=[]  KbParamMax=[]  KtParamMin=[]  KtParamMax=[]  KbOutMin=[]  KbOutMax=[]  KtOutMin=[]  KtOutMax=[]  IntegratorOutMin=[]  IntegratorOutMax=[]  FilterOutMin=[]  FilterOutMax=[]  SumI1OutMin=[]  SumI1OutMax=[]  SumI2OutMin=[]  SumI2OutMax=[]  SumI3OutMin=[]  SumI3OutMax=[]  SumI4OutMin=[]  SumI4OutMax=[]  SumDOutMin=[]  SumDOutMax=[]  DifferentiatorOutMin=[]  DifferentiatorOutMax=[]  FilterDiffOutCoefMin=[]  FilterDiffOutCoefMax=[]  ReciprocalOutMin=[]  ReciprocalOutMax=[]  SumDenOutMin=[]  SumDenOutMax=[]  SumNumOutMin=[]  SumNumOutMax=[]  DivideOutMin=[]  DivideOutMax=[]  UdiffTsProdOutMin=[]  UdiffTsProdOutMax=[]  NTsProdOutMin=[]  NTsProdOutMax=[]  UintegralTsProdOutMin=[]  UintegralTsProdOutMax=[]  UngainTsProdOutMin=[]  UngainTsProdOutMax=[]  ClampingZeroOutDataTypeStr=Inherit: Inherit via back propagation  ClampingZeroOutMin=[]  ClampingZeroOutMax=[]  FilterDenConstantOutDataTypeStr=Inherit: Inherit via back propagation  FilterDenConstantOutMin=[]  FilterDenConstantOutMax=[]  PCopyOutDataTypeStr=Inherit: Inherit via back propagation  PCopyOutMin=[]  PCopyOutMax=[]  NCopyOutDataTypeStr=Inherit: Inherit via back propagation  NCopyOutMin=[]  NCopyOutMax=[]  IntegratorContinuousStateAttributes=''  IntegratorStateMustResolveToSignalObject=off  IntegratorRTWStateStorageClass=Auto  FilterContinuousStateAttributes=''  FilterStateMustResolveToSignalObject=off  FilterRTWStateStorageClass=Auto  ParallelPVariant=InternalParameters  IdealPVariant=Disabled  IVariant=InternalParameters  DVariant=InternalParameters  IntegratorVariant=Continuous  SatVariant=Disabled  AWVariant=Passthrough  PCopyVariant=Disabled  TRVariant=Disabled  FdbkBlocksVariant=Forward  IdealPFdbkVariant=Disabled  SatFdbkVariant=Disabled  DerivativeFilterVariant=ContFilter  NVariant=InternalParameters  NCopyVariant=Disabled  FilterICVariant=InternalICsFilter  IntegratorICVariant=InternalICs  ExternalResetVariant=Disabled  TRSumVariant=Passthrough  SumFdbkVariant=Disabled  SumVariant=Sum_PID  TsampFilterVariant=InternalTs  TsampNgainVariant=Passthrough  TsampIntegralVariant=Disabled_SignalSpec  ExternalSaturationOutDataTypeStr=Inherit: Same as second input
  PID Controller1 : slpidlib/PID Controller  Controller=PID  Form=Parallel  TimeDomain=Continuous-time  UseExternalTs=off  SampleTime=-1  IntegratorMethod=Forward Euler  FilterMethod=Forward Euler  ControllerParametersSource=internal  P=0  I=0  UseKiTs=off  D=0  N=100  UseFilter=on  TunerSelectOption=Transfer Function Based (PID Tuner App)  InitialConditionSource=internal  InitialConditionForIntegrator=0  InitialConditionForFilter=0  DifferentiatorICPrevScaledInput=0  ExternalReset=none  TrackingMode=off  Kt=1  LimitOutput=off  SatLimitsSource=internal  UpperSaturationLimit=inf  LowerSaturationLimit=-inf  LinearizeAsGain=on  AntiWindupMode=none  Kb=1  LimitIntegrator=off  UpperIntegratorSaturationLimit=inf  LowerIntegratorSaturationLimit=-inf  POutMin=[]  POutMax=[]  IOutMin=[]  IOutMax=[]  DOutMin=[]  DOutMax=[]  NOutMin=[]  NOutMax=[]  SumOutMin=[]  SumOutMax=[]  SaturationOutMin=[]  SaturationOutMax=[]  PParamMin=[]  PParamMax=[]  IParamMin=[]  IParamMax=[]  DParamMin=[]  DParamMax=[]  NParamMin=[]  NParamMax=[]  KbParamMin=[]  KbParamMax=[]  KtParamMin=[]  KtParamMax=[]  KbOutMin=[]  KbOutMax=[]  KtOutMin=[]  KtOutMax=[]  IntegratorOutMin=[]  IntegratorOutMax=[]  FilterOutMin=[]  FilterOutMax=[]  SumI1OutMin=[]  SumI1OutMax=[]  SumI2OutMin=[]  SumI2OutMax=[]  SumI3OutMin=[]  SumI3OutMax=[]  SumI4OutMin=[]  SumI4OutMax=[]  SumDOutMin=[]  SumDOutMax=[]  DifferentiatorOutMin=[]  DifferentiatorOutMax=[]  FilterDiffOutCoefMin=[]  FilterDiffOutCoefMax=[]  ReciprocalOutMin=[]  ReciprocalOutMax=[]  SumDenOutMin=[]  SumDenOutMax=[]  SumNumOutMin=[]  SumNumOutMax=[]  DivideOutMin=[]  DivideOutMax=[]  UdiffTsProdOutMin=[]  UdiffTsProdOutMax=[]  NTsProdOutMin=[]  NTsProdOutMax=[]  UintegralTsProdOutMin=[]  UintegralTsProdOutMax=[]  UngainTsProdOutMin=[]  UngainTsProdOutMax=[]  ClampingZeroOutDataTypeStr=Inherit: Inherit via back propagation  ClampingZeroOutMin=[]  ClampingZeroOutMax=[]  FilterDenConstantOutDataTypeStr=Inherit: Inherit via back propagation  FilterDenConstantOutMin=[]  FilterDenConstantOutMax=[]  PCopyOutDataTypeStr=Inherit: Inherit via back propagation  PCopyOutMin=[]  PCopyOutMax=[]  NCopyOutDataTypeStr=Inherit: Inherit via back propagation  NCopyOutMin=[]  NCopyOutMax=[]  IntegratorContinuousStateAttributes=''  IntegratorStateMustResolveToSignalObject=off  IntegratorRTWStateStorageClass=Auto  FilterContinuousStateAttributes=''  FilterStateMustResolveToSignalObject=off  FilterRTWStateStorageClass=Auto  ParallelPVariant=InternalParameters  IdealPVariant=Disabled  IVariant=InternalParameters  DVariant=InternalParameters  IntegratorVariant=Continuous  SatVariant=Disabled  AWVariant=Passthrough  PCopyVariant=Disabled  TRVariant=Disabled  FdbkBlocksVariant=Forward  IdealPFdbkVariant=Disabled  SatFdbkVariant=Disabled  DerivativeFilterVariant=ContFilter  NVariant=InternalParameters  NCopyVariant=Disabled  FilterICVariant=InternalICsFilter  IntegratorICVariant=InternalICs  ExternalResetVariant=Disabled  TRSumVariant=Passthrough  SumFdbkVariant=Disabled  SumVariant=Sum_PID  TsampFilterVariant=InternalTs  TsampNgainVariant=Passthrough  TsampIntegralVariant=Disabled_SignalSpec  ExternalSaturationOutDataTypeStr=Inherit: Same as second input
  Scope{,3..10} (9 alike) : Scope
  Scope1 : Scope  NumInputPorts=2
  Scope2 : Scope  NumInputPorts=2
  Step : Step  Time=0  After=0  SampleTime=0
  Step1 : Step  Time=0  After=0  SampleTime=0
  Sum : Sum  Inputs=|+-
  Sum1 : Sum  Inputs=|+-
  Switch : Switch  Criteria=u2 > Threshold  SaturateOnIntegerOverflow=off  InputSameDT=off
  Switch1 : Switch  Criteria=u2 > Threshold  SaturateOnIntegerOverflow=off  InputSameDT=off
  Terminator : Terminator
  Terminator1 : Terminator
  delta_z : Outport
  delta_y : Outport  Port=2
  wires:
  Demux1/2 -> Scope9/1, [theta_ref]
  Angle_ref/1 -> Demux1/1
  Demux1/3 -> Scope3/1, [psi_ref]
  Angle/1 -> Demux/1
  Demux/3 -> Scope10/1, [psi]
  Demux/2 -> [theta]
  [theta_ref] -> Scope2/1, Sum/1
  [theta] -> Scope2/2, Sum/2
  Demux/1 -> Terminator/1
  Demux1/1 -> Terminator1/1
  [psi_ref] -> Scope1/1, Sum1/1
  [psi] -> Scope1/2, Sum1/2
  Sum/1 -> PID Controller/1
  Sum1/1 -> PID Controller1/1
  Clock/1 -> Compare To Constant/1
  Compare To Constant/1 -> Switch/2
  PID Controller1/1 -> Scope5/1, Switch/1
  Step/1 -> Scope6/1, Switch/3
  Compare To Constant1/1 -> Switch1/2
  Clock1/1 -> Compare To Constant1/1
  PID Controller/1 -> Scope/1, Switch1/1
  Step1/1 -> Scope4/1, Switch1/3
  Switch1/1 -> Scope7/1, delta_y/1
  Switch/1 -> Scope8/1, delta_z/1

== system rocket_sim/TVC模块/F01 ==
  Th : Inport
  F : Inport  Port=2
  Constant7 : Constant  Value=0
  Saturation : Saturate  UpperLimit=1  LowerLimit=0
  Step1 : Step  Time=100  SampleTime=0
  Step2 : Step  Time=300  SampleTime=0
  Switch1 : Switch  Criteria=u2 > Threshold  SaturateOnIntegerOverflow=off  InputSameDT=off
  Switch2 : Switch  Criteria=u2 > Threshold  SaturateOnIntegerOverflow=off  InputSameDT=off
  Switch3 : Switch  Criteria=u2 > Threshold  SaturateOnIntegerOverflow=off  InputSameDT=off
  故障 : Subsystem
  退化 : Subsystem
  Out1 : Outport
  wires:
  Step1/1 -> Switch3/3
  Switch2/1 -> Switch1/3
  Constant7/1 -> Switch3/1
  故障/1(Out1) -> Switch2/1
  退化/1(Out1) -> Switch1/1, Switch2/3
  Th/1 -> 故障/1(Th), 退化/1(Th)
  Switch3/1 -> Switch2/2
  Step2/1 -> Switch1/2
  F/1 -> Switch3/2
  Switch1/1 -> Saturation/1
  Saturation/1 -> Out1/1

== system rocket_sim/TVC模块/Subsystem ==
  Th : Inport
  F : Inport  Port=2
  Constant4 : Constant  Value=0
  Step1 : Step  Time=200  SampleTime=0
  Step2 : Step  Time=480  SampleTime=0
  Switch : Switch  Criteria=u2 > Threshold  SaturateOnIntegerOverflow=off  InputSameDT=off
  Switch1 : Switch  Criteria=u2 > Threshold  SaturateOnIntegerOverflow=off  InputSameDT=off
  Switch2 : Switch  Criteria=u2 > Threshold  SaturateOnIntegerOverflow=off  InputSameDT=off
  故障 : Subsystem
  退化 : Subsystem
  Out1 : Outport
  wires:
  F/1 -> Switch2/2
  退化/1(Out1) -> Switch1/3, Switch/1
  Switch1/1 -> Switch/3
  Constant4/1 -> Switch2/1
  Switch2/1 -> Switch1/2
  Th/1 -> 故障/1(Th1), 退化/1(Th)
  Step2/1 -> Switch/2
  Switch/1 -> Out1/1
  Step1/1 -> Switch2/3
  故障/1(Out1) -> Switch1/1

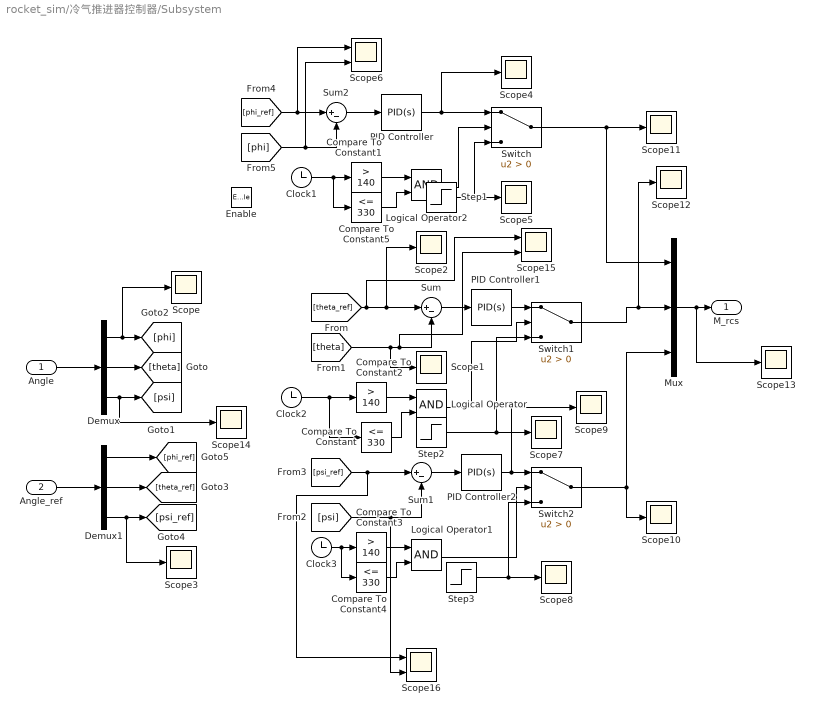
== system rocket_sim/冷气推进器控制器/Subsystem ==
  Angle : Inport
  Angle_ref : Inport  Port=2
  Enable : EnablePort
  Clock1 : Clock
  Clock2 : Clock
  Clock3 : Clock
  Compare To Constant : simulink/Logic and Bit Operations/Compare To Constant  relop=<=  const=330  OutDataTypeStr=boolean
  Compare To Constant1 : simulink/Logic and Bit Operations/Compare To Constant  relop=>  const=140  OutDataTypeStr=boolean
  Compare To Constant2 : simulink/Logic and Bit Operations/Compare To Constant  relop=>  const=140  OutDataTypeStr=boolean
  Compare To Constant3 : simulink/Logic and Bit Operations/Compare To Constant  relop=>  const=140  OutDataTypeStr=boolean
  Compare To Constant4 : simulink/Logic and Bit Operations/Compare To Constant  relop=<=  const=330  OutDataTypeStr=boolean
  Compare To Constant5 : simulink/Logic and Bit Operations/Compare To Constant  relop=<=  const=330  OutDataTypeStr=boolean
  Demux : Demux  Outputs=3
  Demux1 : Demux  Outputs=3
  Logical Operator : Logic  AllPortsSameDT=off  OutDataTypeStr=boolean
  Logical Operator1 : Logic  AllPortsSameDT=off  OutDataTypeStr=boolean
  Logical Operator2 : Logic  AllPortsSameDT=off  OutDataTypeStr=boolean
  Mux : Mux  Inputs=3
  PID Controller : slpidlib/PID Controller  Controller=PID  Form=Parallel  TimeDomain=Continuous-time  UseExternalTs=off  SampleTime=-1  IntegratorMethod=Forward Euler  FilterMethod=Forward Euler  ControllerParametersSource=internal  P=0.002  I=0  UseKiTs=off  D=0.01  N=100  UseFilter=on  TunerSelectOption=Transfer Function Based (PID Tuner App)  InitialConditionSource=internal  InitialConditionForIntegrator=0  InitialConditionForFilter=0  DifferentiatorICPrevScaledInput=0  ExternalReset=none  TrackingMode=off  Kt=1  LimitOutput=off  SatLimitsSource=internal  UpperSaturationLimit=inf  LowerSaturationLimit=-inf  LinearizeAsGain=on  AntiWindupMode=none  Kb=1  LimitIntegrator=off  UpperIntegratorSaturationLimit=inf  LowerIntegratorSaturationLimit=-inf  POutMin=[]  POutMax=[]  IOutMin=[]  IOutMax=[]  DOutMin=[]  DOutMax=[]  NOutMin=[]  NOutMax=[]  SumOutMin=[]  SumOutMax=[]  SaturationOutMin=[]  SaturationOutMax=[]  PParamMin=[]  PParamMax=[]  IParamMin=[]  IParamMax=[]  DParamMin=[]  DParamMax=[]  NParamMin=[]  NParamMax=[]  KbParamMin=[]  KbParamMax=[]  KtParamMin=[]  KtParamMax=[]  KbOutMin=[]  KbOutMax=[]  KtOutMin=[]  KtOutMax=[]  IntegratorOutMin=[]  IntegratorOutMax=[]  FilterOutMin=[]  FilterOutMax=[]  SumI1OutMin=[]  SumI1OutMax=[]  SumI2OutMin=[]  SumI2OutMax=[]  SumI3OutMin=[]  SumI3OutMax=[]  SumI4OutMin=[]  SumI4OutMax=[]  SumDOutMin=[]  SumDOutMax=[]  DifferentiatorOutMin=[]  DifferentiatorOutMax=[]  FilterDiffOutCoefMin=[]  FilterDiffOutCoefMax=[]  ReciprocalOutMin=[]  ReciprocalOutMax=[]  SumDenOutMin=[]  SumDenOutMax=[]  SumNumOutMin=[]  SumNumOutMax=[]  DivideOutMin=[]  DivideOutMax=[]  UdiffTsProdOutMin=[]  UdiffTsProdOutMax=[]  NTsProdOutMin=[]  NTsProdOutMax=[]  UintegralTsProdOutMin=[]  UintegralTsProdOutMax=[]  UngainTsProdOutMin=[]  UngainTsProdOutMax=[]  ClampingZeroOutDataTypeStr=Inherit: Inherit via back propagation  ClampingZeroOutMin=[]  ClampingZeroOutMax=[]  FilterDenConstantOutDataTypeStr=Inherit: Inherit via back propagation  FilterDenConstantOutMin=[]  FilterDenConstantOutMax=[]  PCopyOutDataTypeStr=Inherit: Inherit via back propagation  PCopyOutMin=[]  PCopyOutMax=[]  NCopyOutDataTypeStr=Inherit: Inherit via back propagation  NCopyOutMin=[]  NCopyOutMax=[]  IntegratorContinuousStateAttributes=''  IntegratorStateMustResolveToSignalObject=off  IntegratorRTWStateStorageClass=Auto  FilterContinuousStateAttributes=''  FilterStateMustResolveToSignalObject=off  FilterRTWStateStorageClass=Auto  ParallelPVariant=InternalParameters  IdealPVariant=Disabled  IVariant=InternalParameters  DVariant=InternalParameters  IntegratorVariant=Continuous  SatVariant=Disabled  AWVariant=Passthrough  PCopyVariant=Disabled  TRVariant=Disabled  FdbkBlocksVariant=Forward  IdealPFdbkVariant=Disabled  SatFdbkVariant=Disabled  DerivativeFilterVariant=ContFilter  NVariant=InternalParameters  NCopyVariant=Disabled  FilterICVariant=InternalICsFilter  IntegratorICVariant=InternalICs  ExternalResetVariant=Disabled  TRSumVariant=Passthrough  SumFdbkVariant=Disabled  SumVariant=Sum_PID  TsampFilterVariant=InternalTs  TsampNgainVariant=Passthrough  TsampIntegralVariant=Disabled_SignalSpec  ExternalSaturationOutDataTypeStr=Inherit: Same as second input
  PID Controller1 : slpidlib/PID Controller  Controller=PID  Form=Parallel  TimeDomain=Continuous-time  UseExternalTs=off  SampleTime=-1  IntegratorMethod=Forward Euler  FilterMethod=Forward Euler  ControllerParametersSource=internal  P=0.08  I=0  UseKiTs=off  D=0  N=100  UseFilter=on  TunerSelectOption=Transfer Function Based (PID Tuner App)  InitialConditionSource=internal  InitialConditionForIntegrator=0  InitialConditionForFilter=0  DifferentiatorICPrevScaledInput=0  ExternalReset=none  TrackingMode=off  Kt=1  LimitOutput=off  SatLimitsSource=internal  UpperSaturationLimit=inf  LowerSaturationLimit=-inf  LinearizeAsGain=on  AntiWindupMode=none  Kb=1  LimitIntegrator=off  UpperIntegratorSaturationLimit=inf  LowerIntegratorSaturationLimit=-inf  POutMin=[]  POutMax=[]  IOutMin=[]  IOutMax=[]  DOutMin=[]  DOutMax=[]  NOutMin=[]  NOutMax=[]  SumOutMin=[]  SumOutMax=[]  SaturationOutMin=[]  SaturationOutMax=[]  PParamMin=[]  PParamMax=[]  IParamMin=[]  IParamMax=[]  DParamMin=[]  DParamMax=[]  NParamMin=[]  NParamMax=[]  KbParamMin=[]  KbParamMax=[]  KtParamMin=[]  KtParamMax=[]  KbOutMin=[]  KbOutMax=[]  KtOutMin=[]  KtOutMax=[]  IntegratorOutMin=[]  IntegratorOutMax=[]  FilterOutMin=[]  FilterOutMax=[]  SumI1OutMin=[]  SumI1OutMax=[]  SumI2OutMin=[]  SumI2OutMax=[]  SumI3OutMin=[]  SumI3OutMax=[]  SumI4OutMin=[]  SumI4OutMax=[]  SumDOutMin=[]  SumDOutMax=[]  DifferentiatorOutMin=[]  DifferentiatorOutMax=[]  FilterDiffOutCoefMin=[]  FilterDiffOutCoefMax=[]  ReciprocalOutMin=[]  ReciprocalOutMax=[]  SumDenOutMin=[]  SumDenOutMax=[]  SumNumOutMin=[]  SumNumOutMax=[]  DivideOutMin=[]  DivideOutMax=[]  UdiffTsProdOutMin=[]  UdiffTsProdOutMax=[]  NTsProdOutMin=[]  NTsProdOutMax=[]  UintegralTsProdOutMin=[]  UintegralTsProdOutMax=[]  UngainTsProdOutMin=[]  UngainTsProdOutMax=[]  ClampingZeroOutDataTypeStr=Inherit: Inherit via back propagation  ClampingZeroOutMin=[]  ClampingZeroOutMax=[]  FilterDenConstantOutDataTypeStr=Inherit: Inherit via back propagation  FilterDenConstantOutMin=[]  FilterDenConstantOutMax=[]  PCopyOutDataTypeStr=Inherit: Inherit via back propagation  PCopyOutMin=[]  PCopyOutMax=[]  NCopyOutDataTypeStr=Inherit: Inherit via back propagation  NCopyOutMin=[]  NCopyOutMax=[]  IntegratorContinuousStateAttributes=''  IntegratorStateMustResolveToSignalObject=off  IntegratorRTWStateStorageClass=Auto  FilterContinuousStateAttributes=''  FilterStateMustResolveToSignalObject=off  FilterRTWStateStorageClass=Auto  ParallelPVariant=InternalParameters  IdealPVariant=Disabled  IVariant=InternalParameters  DVariant=InternalParameters  IntegratorVariant=Continuous  SatVariant=Disabled  AWVariant=Passthrough  PCopyVariant=Disabled  TRVariant=Disabled  FdbkBlocksVariant=Forward  IdealPFdbkVariant=Disabled  SatFdbkVariant=Disabled  DerivativeFilterVariant=ContFilter  NVariant=InternalParameters  NCopyVariant=Disabled  FilterICVariant=InternalICsFilter  IntegratorICVariant=InternalICs  ExternalResetVariant=Disabled  TRSumVariant=Passthrough  SumFdbkVariant=Disabled  SumVariant=Sum_PID  TsampFilterVariant=InternalTs  TsampNgainVariant=Passthrough  TsampIntegralVariant=Disabled_SignalSpec  ExternalSaturationOutDataTypeStr=Inherit: Same as second input
  PID Controller2 : slpidlib/PID Controller  Controller=PID  Form=Parallel  TimeDomain=Continuous-time  UseExternalTs=off  SampleTime=-1  IntegratorMethod=Forward Euler  FilterMethod=Forward Euler  ControllerParametersSource=internal  P=0  I=0  UseKiTs=off  D=0  N=100  UseFilter=on  TunerSelectOption=Transfer Function Based (PID Tuner App)  InitialConditionSource=internal  InitialConditionForIntegrator=0  InitialConditionForFilter=0  DifferentiatorICPrevScaledInput=0  ExternalReset=none  TrackingMode=off  Kt=1  LimitOutput=off  SatLimitsSource=internal  UpperSaturationLimit=inf  LowerSaturationLimit=-inf  LinearizeAsGain=on  AntiWindupMode=none  Kb=1  LimitIntegrator=off  UpperIntegratorSaturationLimit=inf  LowerIntegratorSaturationLimit=-inf  POutMin=[]  POutMax=[]  IOutMin=[]  IOutMax=[]  DOutMin=[]  DOutMax=[]  NOutMin=[]  NOutMax=[]  SumOutMin=[]  SumOutMax=[]  SaturationOutMin=[]  SaturationOutMax=[]  PParamMin=[]  PParamMax=[]  IParamMin=[]  IParamMax=[]  DParamMin=[]  DParamMax=[]  NParamMin=[]  NParamMax=[]  KbParamMin=[]  KbParamMax=[]  KtParamMin=[]  KtParamMax=[]  KbOutMin=[]  KbOutMax=[]  KtOutMin=[]  KtOutMax=[]  IntegratorOutMin=[]  IntegratorOutMax=[]  FilterOutMin=[]  FilterOutMax=[]  SumI1OutMin=[]  SumI1OutMax=[]  SumI2OutMin=[]  SumI2OutMax=[]  SumI3OutMin=[]  SumI3OutMax=[]  SumI4OutMin=[]  SumI4OutMax=[]  SumDOutMin=[]  SumDOutMax=[]  DifferentiatorOutMin=[]  DifferentiatorOutMax=[]  FilterDiffOutCoefMin=[]  FilterDiffOutCoefMax=[]  ReciprocalOutMin=[]  ReciprocalOutMax=[]  SumDenOutMin=[]  SumDenOutMax=[]  SumNumOutMin=[]  SumNumOutMax=[]  DivideOutMin=[]  DivideOutMax=[]  UdiffTsProdOutMin=[]  UdiffTsProdOutMax=[]  NTsProdOutMin=[]  NTsProdOutMax=[]  UintegralTsProdOutMin=[]  UintegralTsProdOutMax=[]  UngainTsProdOutMin=[]  UngainTsProdOutMax=[]  ClampingZeroOutDataTypeStr=Inherit: Inherit via back propagation  ClampingZeroOutMin=[]  ClampingZeroOutMax=[]  FilterDenConstantOutDataTypeStr=Inherit: Inherit via back propagation  FilterDenConstantOutMin=[]  FilterDenConstantOutMax=[]  PCopyOutDataTypeStr=Inherit: Inherit via back propagation  PCopyOutMin=[]  PCopyOutMax=[]  NCopyOutDataTypeStr=Inherit: Inherit via back propagation  NCopyOutMin=[]  NCopyOutMax=[]  IntegratorContinuousStateAttributes=''  IntegratorStateMustResolveToSignalObject=off  IntegratorRTWStateStorageClass=Auto  FilterContinuousStateAttributes=''  FilterStateMustResolveToSignalObject=off  FilterRTWStateStorageClass=Auto  ParallelPVariant=InternalParameters  IdealPVariant=Disabled  IVariant=InternalParameters  DVariant=InternalParameters  IntegratorVariant=Continuous  SatVariant=Disabled  AWVariant=Passthrough  PCopyVariant=Disabled  TRVariant=Disabled  FdbkBlocksVariant=Forward  IdealPFdbkVariant=Disabled  SatFdbkVariant=Disabled  DerivativeFilterVariant=ContFilter  NVariant=InternalParameters  NCopyVariant=Disabled  FilterICVariant=InternalICsFilter  IntegratorICVariant=InternalICs  ExternalResetVariant=Disabled  TRSumVariant=Passthrough  SumFdbkVariant=Disabled  SumVariant=Sum_PID  TsampFilterVariant=InternalTs  TsampNgainVariant=Passthrough  TsampIntegralVariant=Disabled_SignalSpec  ExternalSaturationOutDataTypeStr=Inherit: Same as second input
  Scope{,1..5,7..14} (14 alike) : Scope
  Scope15 : Scope  NumInputPorts=2
  Scope16 : Scope  NumInputPorts=2
  Scope6 : Scope  NumInputPorts=2
  Step1 : Step  Time=0  After=0  SampleTime=0
  Step2 : Step  Time=0  After=0  SampleTime=0
  Step3 : Step  Time=0  After=0  SampleTime=0
  Sum : Sum  Inputs=|+-
  Sum1 : Sum  Inputs=|+-
  Sum2 : Sum  Inputs=|+-
  Switch : Switch  Criteria=u2 > Threshold  SaturateOnIntegerOverflow=off  InputSameDT=off
  Switch1 : Switch  Criteria=u2 > Threshold  SaturateOnIntegerOverflow=off  InputSameDT=off
  Switch2 : Switch  Criteria=u2 > Threshold  SaturateOnIntegerOverflow=off  InputSameDT=off
  M_rcs : Outport
  wires:
  Demux1/2 -> [theta_ref]
  Angle_ref/1 -> Demux1/1
  Demux1/3 -> Scope3/1, [psi_ref]
  Angle/1 -> Demux/1
  Demux/3 -> Scope14/1, [psi]
  Demux/2 -> [theta]
  [theta_ref] -> Scope15/1, Scope2/1, Sum/1
  [theta] -> Scope1/1, Scope15/2, Sum/2
  Demux/1 -> Scope/1, [phi]
  [psi_ref] -> Scope16/1, Sum1/1
  [psi] -> Scope16/2, Sum1/2
  Demux1/1 -> [phi_ref]
  [phi_ref] -> Scope6/1, Sum2/1
  [phi] -> Scope6/2, Sum2/2
  Mux/1 -> Scope13/1, M_rcs/1
  Clock1/1 -> Compare To Constant5/1, Compare To Constant1/1
  Step1/1 -> Scope5/1, Switch/3
  Clock2/1 -> Compare To Constant/1, Compare To Constant2/1
  Clock3/1 -> Compare To Constant4/1, Compare To Constant3/1
  Step2/1 -> Scope7/1, Switch1/3
  Step3/1 -> Scope8/1, Switch2/3
  Switch/1 -> Scope11/1, Mux/1
  Switch1/1 -> Scope12/1, Mux/2
  Switch2/1 -> Mux/3, Scope10/1
  Sum2/1 -> PID Controller/1
  PID Controller/1 -> Scope4/1, Switch/1
  PID Controller1/1 -> Switch1/1
  Sum/1 -> PID Controller1/1
  PID Controller2/1 -> Scope9/1, Switch2/1
  Sum1/1 -> PID Controller2/1
  Compare To Constant2/1 -> Logical Operator/1
  Logical Operator/1 -> Switch1/2
  Compare To Constant/1 -> Logical Operator/2
  Compare To Constant3/1 -> Logical Operator1/1
  Logical Operator1/1 -> Switch2/2
  Compare To Constant4/1 -> Logical Operator1/2
  Compare To Constant1/1 -> Logical Operator2/1
  Logical Operator2/1 -> Switch/2
  Compare To Constant5/1 -> Logical Operator2/2

== system rocket_sim/冷气推进器控制器/Subsystem1 ==
  Th : Inport
  F : Inport  Port=2
  Constant4 : Constant  Value=0
  Step1 : Step  Time=200  SampleTime=0
  Step2 : Step  Time=480  SampleTime=0
  Switch : Switch  Criteria=u2 > Threshold  SaturateOnIntegerOverflow=off  InputSameDT=off
  Switch1 : Switch  Criteria=u2 > Threshold  SaturateOnIntegerOverflow=off  InputSameDT=off
  Switch2 : Switch  Criteria=u2 > Threshold  SaturateOnIntegerOverflow=off  InputSameDT=off
  故障 : Subsystem
  退化 : Subsystem
  Out1 : Outport
  wires:
  F/1 -> Switch2/2
  退化/1(Out1) -> Switch1/3, Switch/1
  Switch1/1 -> Switch/3
  Constant4/1 -> Switch2/1
  Switch2/1 -> Switch1/2
  Th/1 -> 故障/1(Th1), 退化/1(Th)
  Step2/1 -> Switch/2
  Switch/1 -> Out1/1
  Step1/1 -> Switch2/3
  故障/1(Out1) -> Switch1/1
